simulink model "demo_fim_replacements"  (R2026a)
settings: Solver=FixedStepDiscrete  StopTime=7  FixedStep=1
settings Model: Creator=harry_31916  LastModifiedBy=harry_31916
settings OptimizationCC: BooleanDataType=off

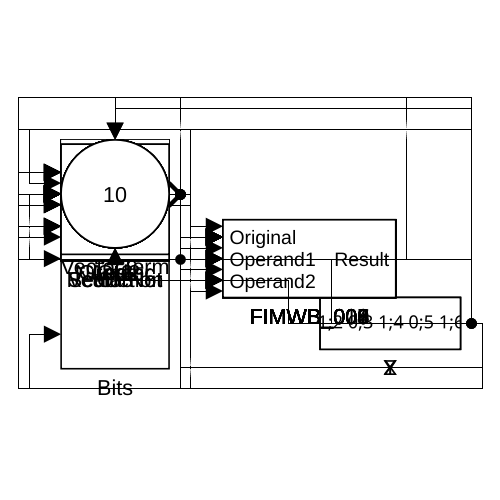
[thumbnail: Simulink's stored preview of the top-level diagram]
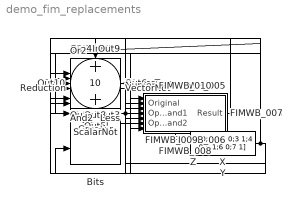
== system demo_fim_replacements ==
  And2 : Logic  AllPortsSameDT=off  OutDataTypeStr=boolean
  Bits : Mux  Inputs=3
  FIMWB_001 : Subsystem  Tag=fimwb.fault.1
  FIMWB_002 : Subsystem  Tag=fimwb.fault.2
  FIMWB_003 : Subsystem  Tag=fimwb.fault.3
  FIMWB_004 : Subsystem  Tag=fimwb.fault.4
  FIMWB_005 : Subsystem  Tag=fimwb.fault.5
  FIMWB_006 : Subsystem  Tag=fimwb.fault.6
  FIMWB_007 : Subsystem  Tag=fimwb.fault.7
  FIMWB_008 : Subsystem  Tag=fimwb.fault.8
  FIMWB_009 : Subsystem  Tag=fimwb.fault.9
  FIMWB_010 : Subsystem  Tag=fimwb.fault.10
  Greater : RelationalOperator  Operator=>
  Less : RelationalOperator  Operator=<
  Minus : Sum  Inputs=--
  Numeric : Logic  Operator=OR  AllPortsSameDT=off
  Or2 : Logic  Operator=OR  AllPortsSameDT=off  OutDataTypeStr=boolean
  Or3 : Logic  Operator=OR  Inputs=3  AllPortsSameDT=off  OutDataTypeStr=boolean
  Plus : Sum
  Reduction : Logic  Inputs=1  AllPortsSameDT=off  OutDataTypeStr=boolean
  ScalarNot : Logic  Operator=NOT  Inputs=1  AllPortsSameDT=off  OutDataTypeStr=boolean
  VectorNot : Logic  Operator=NOT  Inputs=1  AllPortsSameDT=off  OutDataTypeStr=boolean
  VectorTerm : Terminator
  X : FromWorkspace  VariableName=[0 0;1 0;2 0;3 0;4 -2;5 -2;6 2;7 2]  SampleTime=1  Interpolate=off  OutputAfterFinalValue=Holding final value
  XBool : DataTypeConversion  OutDataTypeStr=boolean
  XInt : DataTypeConversion  OutDataTypeStr=int16
  Y : FromWorkspace  VariableName=[0 0;1 0;2 3;3 3;4 0;5 0;6 1;7 1]  SampleTime=1  Interpolate=off  OutputAfterFinalValue=Holding final value
  YBool : DataTypeConversion  OutDataTypeStr=boolean
  YInt : DataTypeConversion  OutDataTypeStr=int16
  Z : FromWorkspace  VariableName=[0 0;1 1;2 0;3 1;4 0;5 1;6 0;7 1]  SampleTime=1  Interpolate=off  OutputAfterFinalValue=Holding final value
  ZBool : DataTypeConversion  OutDataTypeStr=boolean
  ZInt : DataTypeConversion  OutDataTypeStr=int16
  Out1 : Outport
  Out2 : Outport  Port=2
  Out3 : Outport  Port=3
  Out4 : Outport  Port=4
  Out5 : Outport  Port=5
  Out6 : Outport  Port=6
  Out7 : Outport  Port=7
  Out8 : Outport  Port=8
  Out9 : Outport  Port=9
  Out10 : Outport  Port=10
  wires:
  X/1 -> XBool/1, XInt/1, Numeric/1, Plus/1, Minus/1, FIMWB_004/2(Operand1), FIMWB_009/2(Operand1), FIMWB_010/2(Operand1)
  Y/1 -> YBool/1, YInt/1, Numeric/2, Plus/2, Minus/2, FIMWB_004/3(Operand2), FIMWB_009/3(Operand2), FIMWB_010/3(Operand2)
  Z/1 -> ZBool/1, ZInt/1
  XBool/1 -> Bits/1, And2/1, Or2/1, Or3/1, ScalarNot/1, FIMWB_001/2(Operand1), FIMWB_002/2(Operand1), FIMWB_003/2(Operand1), FIMWB_006/2(Operand1)
  YBool/1 -> Bits/2, And2/2, Or2/2, Or3/2, FIMWB_001/3(Operand2), FIMWB_002/3(Operand2), FIMWB_003/3(Operand2)
  ZBool/1 -> Bits/3, Or3/3, FIMWB_003/4(Operand3)
  Bits/1 -> Reduction/1, VectorNot/1, FIMWB_005/2(Operand1)
  VectorNot/1 -> VectorTerm/1
  XInt/1 -> Greater/1, Less/1, FIMWB_007/2(Operand1), FIMWB_008/2(Operand1)
  YInt/1 -> Greater/2, Less/2, FIMWB_007/3(Operand2), FIMWB_008/3(Operand2)
  And2/1 -> FIMWB_001/1(Original)
  FIMWB_001/1(Result) -> Out1/1
  Or2/1 -> FIMWB_002/1(Original)
  FIMWB_002/1(Result) -> Out2/1
  Or3/1 -> FIMWB_003/1(Original)
  FIMWB_003/1(Result) -> Out3/1
  Numeric/1 -> FIMWB_004/1(Original)
  FIMWB_004/1(Result) -> Out4/1
  Reduction/1 -> FIMWB_005/1(Original)
  FIMWB_005/1(Result) -> Out5/1
  ScalarNot/1 -> FIMWB_006/1(Original)
  FIMWB_006/1(Result) -> Out6/1
  Greater/1 -> FIMWB_007/1(Original)
  FIMWB_007/1(Result) -> Out7/1
  Less/1 -> FIMWB_008/1(Original)
  FIMWB_008/1(Result) -> Out8/1
  Plus/1 -> FIMWB_009/1(Original)
  FIMWB_009/1(Result) -> Out9/1
  Minus/1 -> FIMWB_010/1(Original)
  FIMWB_010/1(Result) -> Out10/1

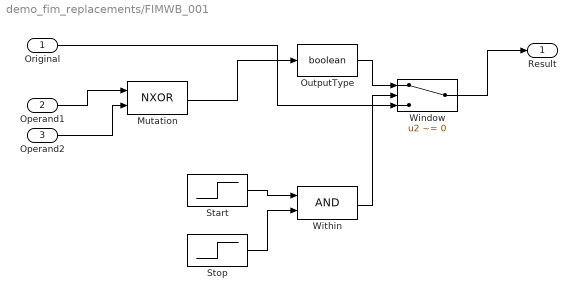
== system demo_fim_replacements/FIMWB_001 ==
  Original : Inport
  Operand1 : Inport  Port=2
  Operand2 : Inport  Port=3
  Mutation : Logic  Operator=NXOR  AllPortsSameDT=off  OutDataTypeStr=boolean
  OutputType : DataTypeConversion  OutDataTypeStr=boolean  RndMeth=Round
  Start : Step  Time=2  SampleTime=0
  Stop : Step  Time=6  InitialValue=1  FinalValue=0  SampleTime=0
  Window : Switch  Criteria=u2 ~= 0  SaturateOnIntegerOverflow=off  InputSameDT=off
  Within : Logic  AllPortsSameDT=off  OutDataTypeStr=boolean
  Result : Outport
  wires:
  Operand1/1 -> Mutation/1
  Operand2/1 -> Mutation/2
  Mutation/1 -> OutputType/1
  Start/1 -> Within/1
  Stop/1 -> Within/2
  OutputType/1 -> Window/1
  Within/1 -> Window/2
  Original/1 -> Window/3
  Window/1 -> Result/1

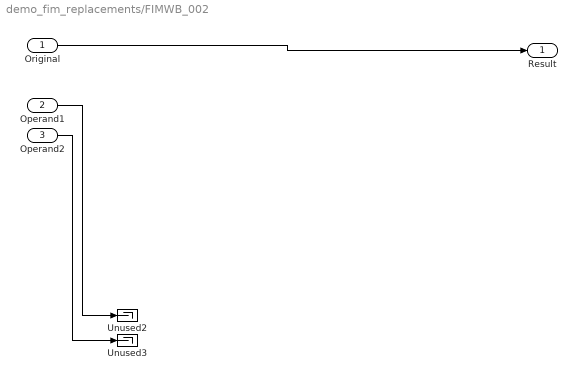
== system demo_fim_replacements/FIMWB_002 ==
  Original : Inport
  Operand1 : Inport  Port=2
  Operand2 : Inport  Port=3
  Unused2 : Terminator
  Unused3 : Terminator
  Result : Outport
  wires:
  Original/1 -> Result/1
  Operand1/1 -> Unused2/1
  Operand2/1 -> Unused3/1

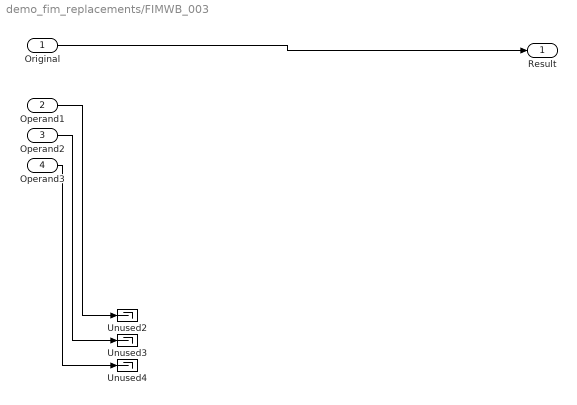
== system demo_fim_replacements/FIMWB_003 ==
  Original : Inport
  Operand1 : Inport  Port=2
  Operand2 : Inport  Port=3
  Operand3 : Inport  Port=4
  Unused2 : Terminator
  Unused3 : Terminator
  Unused4 : Terminator
  Result : Outport
  wires:
  Original/1 -> Result/1
  Operand1/1 -> Unused2/1
  Operand2/1 -> Unused3/1
  Operand3/1 -> Unused4/1

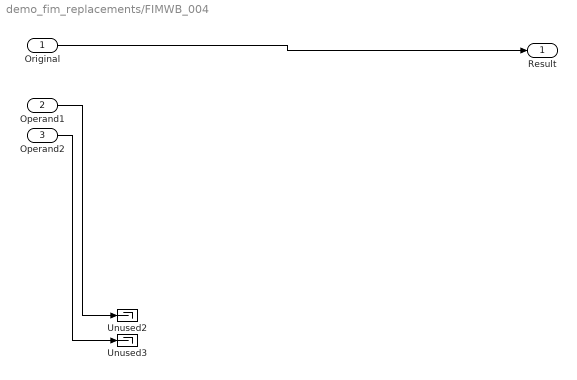
== system demo_fim_replacements/FIMWB_004 ==
  Original : Inport
  Operand1 : Inport  Port=2
  Operand2 : Inport  Port=3
  Unused2 : Terminator
  Unused3 : Terminator
  Result : Outport
  wires:
  Original/1 -> Result/1
  Operand1/1 -> Unused2/1
  Operand2/1 -> Unused3/1

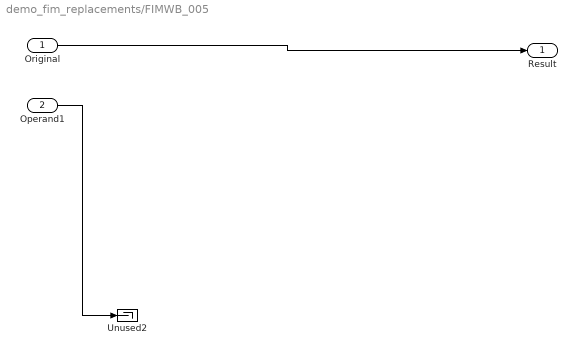
== system demo_fim_replacements/FIMWB_005 ==
  Original : Inport
  Operand1 : Inport  Port=2
  Unused2 : Terminator
  Result : Outport
  wires:
  Original/1 -> Result/1
  Operand1/1 -> Unused2/1

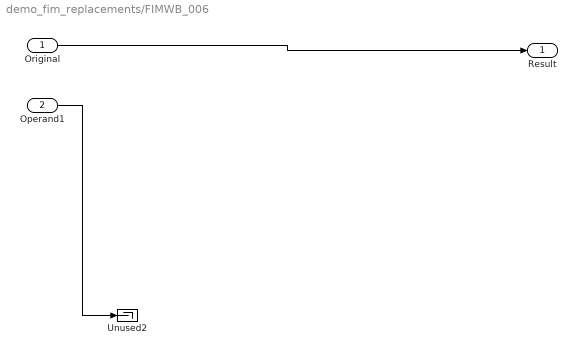
== system demo_fim_replacements/FIMWB_006 ==
  Original : Inport
  Operand1 : Inport  Port=2
  Unused2 : Terminator
  Result : Outport
  wires:
  Original/1 -> Result/1
  Operand1/1 -> Unused2/1

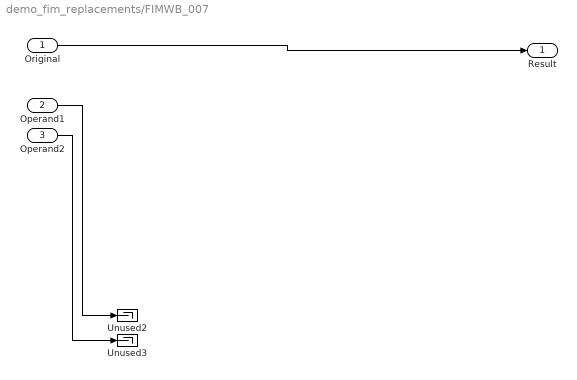
== system demo_fim_replacements/FIMWB_007 ==
  Original : Inport
  Operand1 : Inport  Port=2
  Operand2 : Inport  Port=3
  Unused2 : Terminator
  Unused3 : Terminator
  Result : Outport
  wires:
  Original/1 -> Result/1
  Operand1/1 -> Unused2/1
  Operand2/1 -> Unused3/1

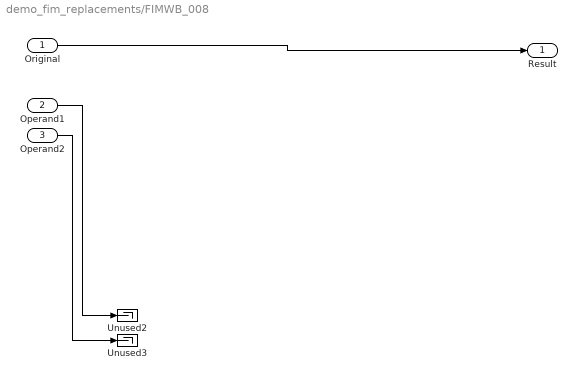
== system demo_fim_replacements/FIMWB_008 ==
  Original : Inport
  Operand1 : Inport  Port=2
  Operand2 : Inport  Port=3
  Unused2 : Terminator
  Unused3 : Terminator
  Result : Outport
  wires:
  Original/1 -> Result/1
  Operand1/1 -> Unused2/1
  Operand2/1 -> Unused3/1

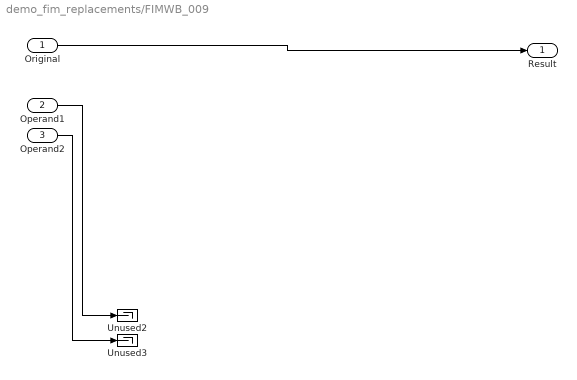
== system demo_fim_replacements/FIMWB_009 ==
  Original : Inport
  Operand1 : Inport  Port=2
  Operand2 : Inport  Port=3
  Unused2 : Terminator
  Unused3 : Terminator
  Result : Outport
  wires:
  Original/1 -> Result/1
  Operand1/1 -> Unused2/1
  Operand2/1 -> Unused3/1

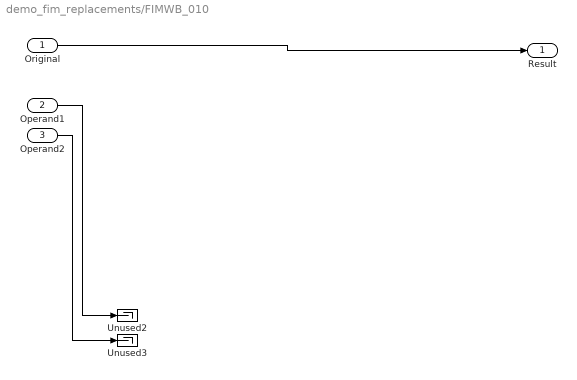
== system demo_fim_replacements/FIMWB_010 ==
  Original : Inport
  Operand1 : Inport  Port=2
  Operand2 : Inport  Port=3
  Unused2 : Terminator
  Unused3 : Terminator
  Result : Outport
  wires:
  Original/1 -> Result/1
  Operand1/1 -> Unused2/1
  Operand2/1 -> Unused3/1
